simulink model "Simulateur_palan_generateur_trajectoire"  (R2026a)
settings: Solver=ode4  StopTime=20
values from neighbouring files (symbols this model uses):
  F = sysd.A    [Script_projet_section2.m]    (also in labo6_simulation.m)
  G = 0.002    [Essai_boucle_ouverte.mat]    (also in PAR_PAL1_IDENT.m; Script_projet_section2.m = sysd.B; labo6_simulation.m = sysd.B; mncarres_incomplet.m)
  Kr = [0.1 0 0 0]    [Essai_boucle_ouverte.mat]    (also in Script_projet_section2.m = [9.0560    4.5832  -13.7344    0.1]; labo6_simulation.m = [9.9952 2.8361 -8.7562 1.2009])
  L = 0.1    [ETAT_PAL_IDENT.m]    (also in Essai_boucle_ouverte.mat; Script_projet_section2.m = 1; labo6_simulation.m; p1_cre_18V_droite_0m.mat = 0)
  xd_ref = 0.5    [Script_projet_section2.m]    (also in labo6_simulation.m)
libraries: cstblocks_lti x2
settings Model: Creator=Ale  LastModifiedBy=justi

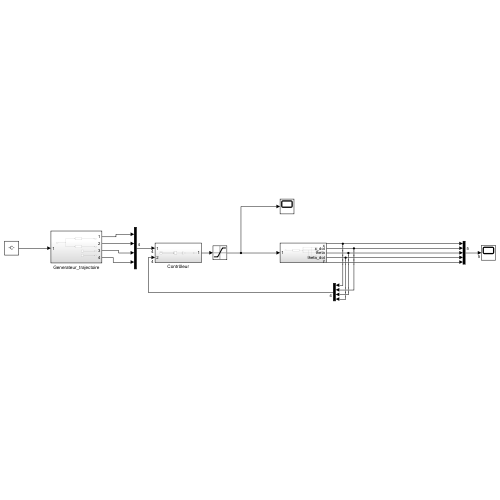
[thumbnail: Simulink's stored preview of the top-level diagram]
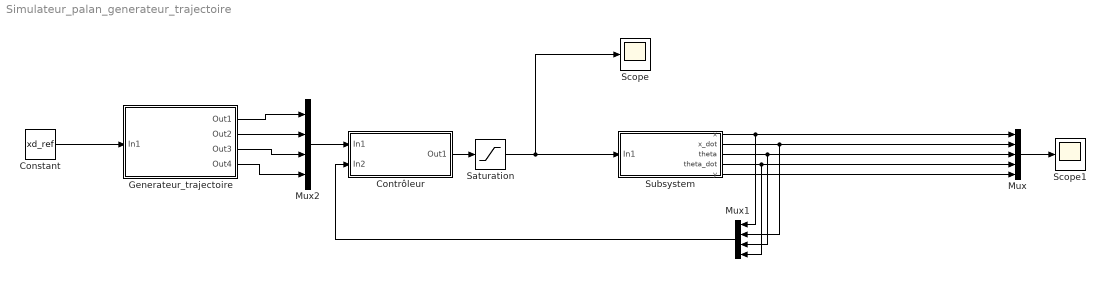
== system Simulateur_palan_generateur_trajectoire ==
  Constant : Constant  Value=xd_ref
  Contrôleur : Subsystem
  Generateur_trajectoire : Subsystem
  Mux : Mux  Inputs=5
  Mux1 : Mux
  Mux2 : Mux
  Saturation : Saturate  UpperLimit=24  LowerLimit=-24
  Scope : Scope
      settings: ActiveDisplayYMinimum=0.058367510547742807  ActiveDisplayYMaximum=1.577089384081257  DataLoggingSaveFormat=Array
  Scope1 : Scope
      settings: ActiveDisplayYMinimum=-0.27018718362053207  ActiveDisplayYMaximum=0.733930627828778  DataLoggingSaveFormat=Array
  Subsystem : Subsystem
  wires:
  Subsystem/1(x) -> Mux1/1, Mux/1
  Subsystem/2(x_dot) -> Mux1/2, Mux/2
  Subsystem/3(theta) -> Mux1/3, Mux/3
  Subsystem/4(theta_dot) -> Mux1/4, Mux/4
  Subsystem/5(y) -> Mux/5
  Mux/1 -> Scope1/1
  Mux1/1 -> Contrôleur/2(In2)
  Contrôleur/1(Out1) -> Saturation/1
  Saturation/1 -> Scope/1, Subsystem/1(In1)
  Mux2/1 -> Contrôleur/1(In1)
  Generateur_trajectoire/1(Out1) -> Mux2/1
  Generateur_trajectoire/2(Out2) -> Mux2/2
  Generateur_trajectoire/3(Out3) -> Mux2/3
  Generateur_trajectoire/4(Out4) -> Mux2/4
  Constant/1 -> Generateur_trajectoire/1(In1)

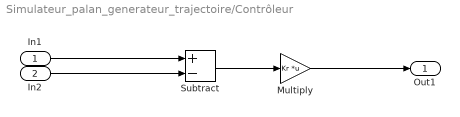
== system Simulateur_palan_generateur_trajectoire/Contrôleur ==
  In1 : Inport
  In2 : Inport  Port=2
  Multiply : Gain  Gain=Kr  Multiplication=Matrix(K*u)
  Subtract : Sum  Inputs=+-
  Out1 : Outport
  wires:
  In1/1 -> Subtract/1
  In2/1 -> Subtract/2
  Subtract/1 -> Multiply/1
  Multiply/1 -> Out1/1

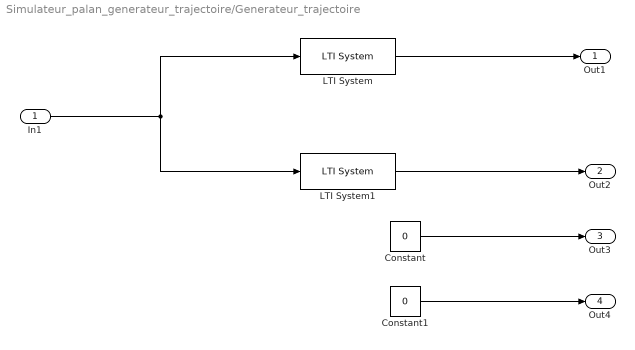
== system Simulateur_palan_generateur_trajectoire/Generateur_trajectoire ==
  In1 : Inport
  Constant : Constant  Value=0
  Constant1 : Constant  Value=0
  LTI System : cstblocks_lti/LTI System  sys=H_pos_d  IC=[]  PadeOrder=0
      settings: LibrarySourceBlock=cstblocks/LTI System
  LTI System1 : cstblocks_lti/LTI System  sys=H_vit_d  IC=[]  PadeOrder=0
      settings: LibrarySourceBlock=cstblocks/LTI System
  Out1 : Outport
  Out2 : Outport  Port=2
  Out3 : Outport  Port=3
  Out4 : Outport  Port=4
  wires:
  In1/1 -> LTI System/1, LTI System1/1
  LTI System/1 -> Out1/1
  LTI System1/1 -> Out2/1
  Constant/1 -> Out3/1
  Constant1/1 -> Out4/1

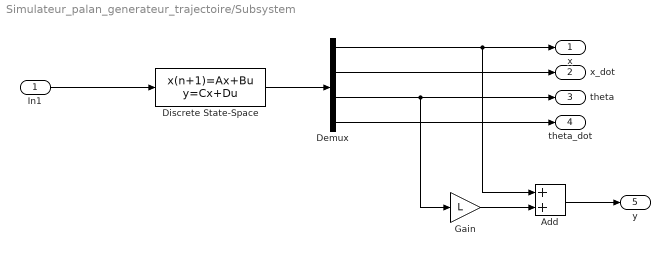
== system Simulateur_palan_generateur_trajectoire/Subsystem ==
  In1 : Inport
  Add : Sum
  Demux : Demux
  Discrete State-Space : DiscreteStateSpace  A=F  B=G  C=[1 0 0 0;0 1 0 0; 0 0 1 0; 0 0 0 1]  D=[0;0;0;0]  SampleTime=-1
  Gain : Gain  Gain=L
  x : Outport
  x_dot : Outport  Port=2
  theta : Outport  Port=3
  theta_dot : Outport  Port=4
  y : Outport  Port=5
  wires:
  Demux/2 -> x_dot/1
  Demux/1 -> x/1, Add/1
  Demux/4 -> theta_dot/1
  Demux/3 -> theta/1, Gain/1
  Gain/1 -> Add/2
  Add/1 -> y/1
  In1/1 -> Discrete State-Space/1
  Discrete State-Space/1 -> Demux/1
